simulink model "Open_loop_speed_control_of_PMSM_drive"  (R2024a)
settings: Solver=ode4  StartTime=0.0  StopTime=0.5  FixedStep=1e-5  RelTol=1e-3
libraries: spsIGBTDiodeLib x6, spsDCVoltageSourceLib x1, spsPermanentMagnetSynchronousMachineLib x1, simulink x1, spsThreePhaseVIMeasurementLib x1, sps_lib x1
settings Model: Creator=DINAKAR  LastModifiedBy=haris

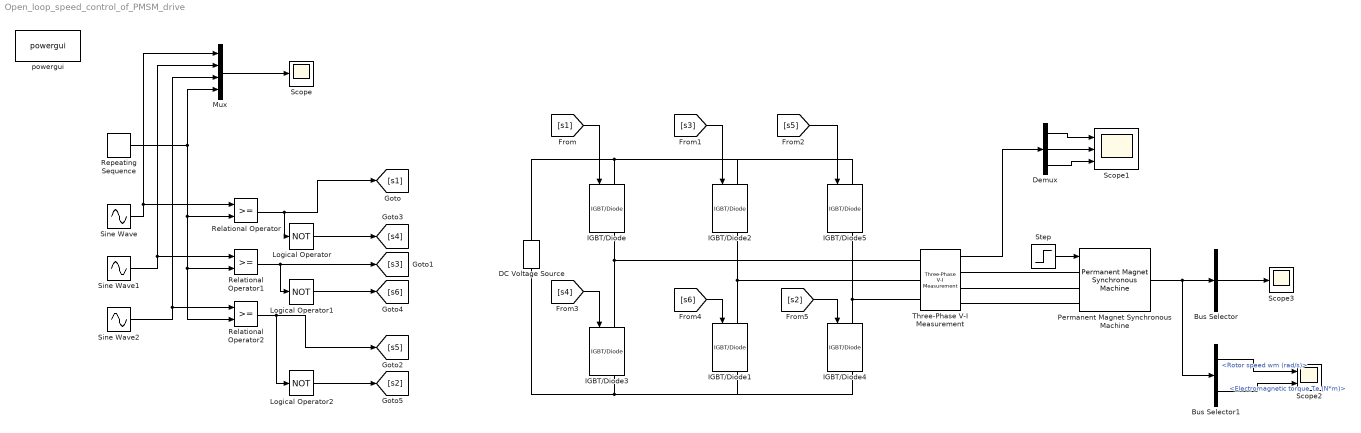
== system Open_loop_speed_control_of_PMSM_drive ==
  Bus Selector : BusSelector  OutputSignals=Stator current is_a (A),Stator current is_b (A),Stator current is_c (A)  OutputAsBus=on
  Bus Selector1 : BusSelector  OutputSignals=Rotor speed wm (rad/s),Electromagnetic torque Te (N*m)
  DC Voltage Source : spsDCVoltageSourceLib/DC Voltage Source  Amplitude=400  Measurements=None
  Demux : Demux  Outputs=3
  IGBT/Diode{,1..5} (6 alike) : spsIGBTDiodeLib/IGBT//Diode  Ron=1e-3  Rs=1e5  Cs=inf  Measurements=on
  Logical Operator : Logic  Operator=NOT  AllPortsSameDT=off  OutDataTypeStr=boolean
  Logical Operator1 : Logic  Operator=NOT  AllPortsSameDT=off  OutDataTypeStr=boolean
  Logical Operator2 : Logic  Operator=NOT  AllPortsSameDT=off  OutDataTypeStr=boolean
  Mux : Mux
  Permanent Magnet Synchronous Machine : spsPermanentMagnetSynchronousMachineLib/Permanent Magnet Synchronous Machine  NbPhases=3  FluxDistribution=Sinusoidal  RotorType=Round  MechanicalLoad=Torque Tm  PresetModel="02:  1.7 Nm 300 Vdc 3750 RPM - 1.7 Nm"  ShowDetailedParameters=on  MeasurementBus=off  Resistance=4.765  Inductance=8.5e-3  dqInductances=[8.5e-3,8.5e-3]  La=0.014  MachineConstant=Flux linkage established by magnets (V.s)  Flux=0.1848  VoltageCst=67.038  TorqueCst=0.5544  Flat=120  Mechanical=[0.0001051 4.047e-05 2 0]  PolePairs=2  InitialConditions=[0,0, 0,0]  InitialConditions5ph=[0 0 0 0 0 0]  RefAngle=90 degrees behind phase A axis (modified Park)  IterativeDiscreteModel=Trapezoidal non iterative  TsBlock=-1  TsPowergui=0
  Relational Operator : RelationalOperator  OutDataTypeStr=boolean  RndMeth=Simplest  InputSameDT=off
  Relational Operator1 : RelationalOperator  OutDataTypeStr=boolean  RndMeth=Simplest  InputSameDT=off
  Relational Operator2 : RelationalOperator  OutDataTypeStr=boolean  RndMeth=Simplest  InputSameDT=off
  Repeating Sequence : simulink/Sources/Repeating Sequence  rep_seq_t=[0 1 2 3]*[1/6000]  rep_seq_y=[0 1 -1 0]
  Scope : Scope
  Scope1 : Scope  NumInputPorts=3
  Scope2 : Scope  NumInputPorts=2
  Scope3 : Scope
  Sine Wave : Sin  Frequency=2*pi*50  SampleTime=0
  Sine Wave1 : Sin  Frequency=2*pi*50  Phase=4*pi/3  SampleTime=0
  Sine Wave2 : Sin  Frequency=2*pi*50  Phase=2*pi/3  SampleTime=0
  Step : Step  Time=0.2  Before=1  After=3  SampleTime=0
  Three-Phase V-I Measurement : spsThreePhaseVIMeasurementLib/Three-Phase V-I Measurement  VoltageMeasurement=phase-to-phase  SetLabelV=off  LabelV=Vabc  Vpu=off  VpuLL=off  CurrentMeasurement=no  SetLabelI=off  LabelI=Iabc  Ipu=off  Pbase=100e6  Vbase=500e3  OutputType=Complex  PhasorSimulation=off  PSBequivalent=0
  powergui : sps_lib/powergui  Priority=1  SimulationMode=Continuous  SampleTime=50e-6  frequency=60  Iterations=50  frequencyindice=0  Pbase=100e6  ErrMax=1e-4  UnitsV=kV  UnitsW=MW  buscounter=0  FunctionMessages=off  echomessages=off  EnableUseOfTLC=off  CurrentSourceSwitches=off  DisableSnubberDevices=off  DisableRonSwitches=off  DisableVfSwitches=off  DisplayEquations=off  AutomaticDiscreteSolvers=off  SolverType=Tustin/Backward Euler (TBE)  Interpol=off  ExternalGateDelay=off  methode=off  Ts=100  x0status=blocks  SPID=on  SwTol=0  HookPort=off  NonlinearTolerance=1e-4  nMaxIteration=100  ContinueOnMaxIteration=off  RestoreLinks=warning  ResistiveCurrentMeasurement=off  Frange=[0:2:500]  Ylog=off  Xlog=on  ShowGrid=off  save=off  variable=ZData  structure=0  ZoomFFT=off  StartTime=0.0  cycles=1  DisplayStyle=1  fundamental=60  FreqAxis=off  MaxFrequency=1000  frequencyindicesteady=1  RmsSteady=1  display=off
  wires:
  Repeating Sequence/1 -> Mux/4, Relational Operator1/2, Relational Operator2/2, Relational Operator/2
  Sine Wave/1 -> Mux/1, Relational Operator/1
  Sine Wave1/1 -> Mux/2, Relational Operator1/1
  Sine Wave2/1 -> Mux/3, Relational Operator2/1
  Mux/1 -> Scope/1
  Relational Operator2/1 -> [s5], Logical Operator2/1
  Relational Operator1/1 -> Logical Operator1/1, [s3]
  Relational Operator/1 -> Logical Operator/1, [s1]
  Logical Operator/1 -> [s4]
  Logical Operator1/1 -> [s6]
  Logical Operator2/1 -> [s2]
  [s5] -> IGBT/Diode5/1
  [s3] -> IGBT/Diode2/1
  [s1] -> IGBT/Diode/1
  [s2] -> IGBT/Diode4/1
  [s6] -> IGBT/Diode1/1
  [s4] -> IGBT/Diode3/1
  Demux/2 -> Scope1/2
  Demux/1 -> Scope1/1
  Demux/3 -> Scope1/3
  Three-Phase V-I Measurement/1 -> Demux/1
  Bus Selector1/1 -> Scope2/1  "<Rotor speed wm (rad/s)>"
  Bus Selector1/2 -> Scope2/2  "<Electromagnetic torque Te (N*m)>"
  Bus Selector/1 -> Scope3/1
  Step/1 -> Permanent Magnet Synchronous Machine/1
  Permanent Magnet Synchronous Machine/1 -> Bus Selector/1, Bus Selector1/1
  connections:
  DC Voltage Source/RConn1 -- IGBT/Diode5/LConn1 -- IGBT/Diode2/LConn1 -- IGBT/Diode/LConn1
  IGBT/Diode3/RConn1 -- IGBT/Diode4/RConn1 -- IGBT/Diode1/RConn1 -- DC Voltage Source/LConn1
  IGBT/Diode5/RConn1 -- Three-Phase V-I Measurement/LConn3 -- IGBT/Diode4/LConn1
  IGBT/Diode/RConn1 -- Three-Phase V-I Measurement/LConn1 -- IGBT/Diode3/LConn1
  IGBT/Diode2/RConn1 -- Three-Phase V-I Measurement/LConn2 -- IGBT/Diode1/LConn1
  Permanent Magnet Synchronous Machine/LConn1 -- Three-Phase V-I Measurement/RConn1
  Three-Phase V-I Measurement/RConn2 -- Permanent Magnet Synchronous Machine/LConn2
  Three-Phase V-I Measurement/RConn3 -- Permanent Magnet Synchronous Machine/LConn3
